simulink model "Example"  (R2026a)
settings: Solver=VariableStepAuto
settings Model: Creator=aleck  LastModifiedBy=aleck

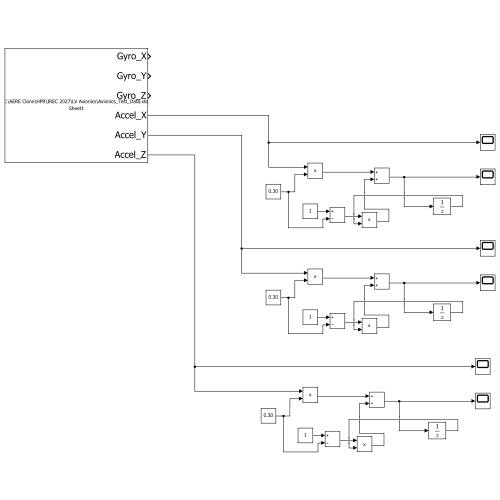
[thumbnail: Simulink's stored preview of the top-level diagram]
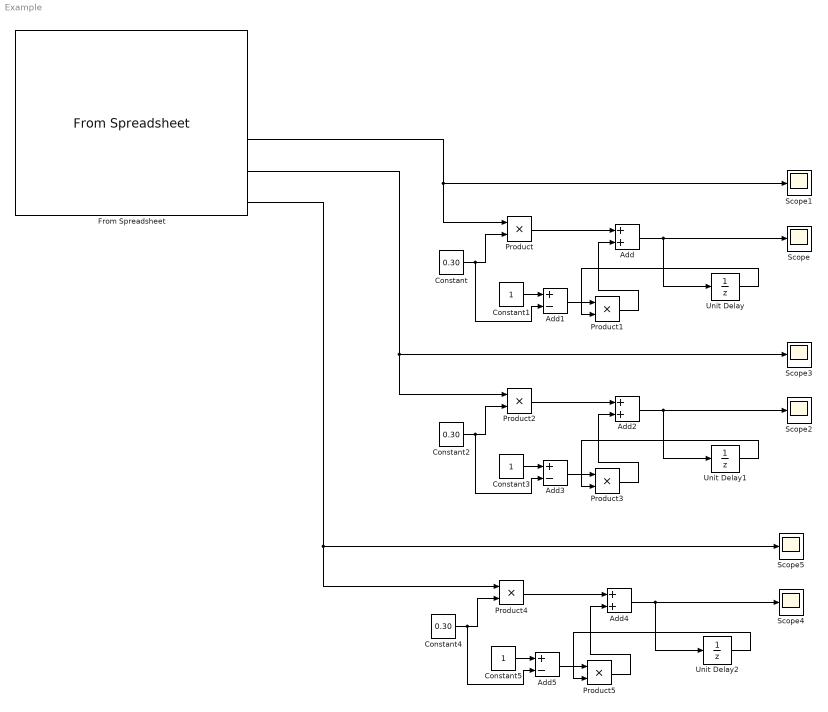
== system Example ==
  Add : Sum
  Add1 : Sum  Inputs=+-
  Add2 : Sum
  Add3 : Sum  Inputs=+-
  Add4 : Sum
  Add5 : Sum  Inputs=+-
  Constant : Constant  Value=0.30
  Constant1 : Constant
  Constant2 : Constant  Value=0.30
  Constant3 : Constant
  Constant4 : Constant  Value=0.30
  Constant5 : Constant
  From Spreadsheet : FromSpreadsheet  FileName=C:\AERE Clone\HPR\IREC 2027\LV Avionics\Avionics_Test_Data.xlsx  Range=A1:G31014  SampleTime=0.002
  Product{,1..5} (6 alike) : Product
  Scope{,1..5} (6 alike) : Scope
      Scope settings: ActiveDisplayYMinimum=-24.187789382642912  ActiveDisplayYMaximum=12.941672746916071
      Scope1 settings: ActiveDisplayYMinimum=-2.1640960629111281  ActiveDisplayYMaximum=2.9077671265449037
      Scope2 settings: ActiveDisplayYMinimum=-0.575153452596094  ActiveDisplayYMaximum=0.40171119344323236  DataLoggingVariableName=ScopeData2
      Scope3 settings: ActiveDisplayYMinimum=-0.23912409618807512  ActiveDisplayYMaximum=0.31406317313425119  DataLoggingVariableName=ScopeData3
      Scope4 settings: ActiveDisplayYMinimum=-0.17738138422278368  ActiveDisplayYMaximum=0.24432598614259191  DataLoggingVariableName=ScopeData4
      Scope5 settings: ActiveDisplayYMinimum=0.031018770222674557  ActiveDisplayYMaximum=0.079724381908564526  DataLoggingVariableName=ScopeData5
  Unit Delay : UnitDelay  SampleTime=-1
  Unit Delay1 : UnitDelay  SampleTime=-1
  Unit Delay2 : UnitDelay  SampleTime=-1
  wires:
  From Spreadsheet/4 -> Product/1, Scope1/1
  Constant/1 -> Add1/2, Product/2
  Product/1 -> Add/1
  Constant1/1 -> Add1/1
  Add1/1 -> Product1/1
  Unit Delay/1 -> Product1/2
  Product1/1 -> Add/2
  Add/1 -> Unit Delay/1, Scope/1
  Product3/1 -> Add2/2
  Product2/1 -> Add2/1
  Constant2/1 -> Add3/2, Product2/2
  Add2/1 -> Unit Delay1/1, Scope2/1
  Constant3/1 -> Add3/1
  Add3/1 -> Product3/1
  Unit Delay1/1 -> Product3/2
  Constant5/1 -> Add5/1
  Add4/1 -> Unit Delay2/1, Scope4/1
  Add5/1 -> Product5/1
  Constant4/1 -> Add5/2, Product4/2
  Product4/1 -> Add4/1
  Product5/1 -> Add4/2
  Unit Delay2/1 -> Product5/2
  From Spreadsheet/5 -> Product2/1, Scope3/1
  From Spreadsheet/6 -> Scope5/1, Product4/1
